simulink model "TEPC_Electronics"  (R2025a)
settings: Solver=FixedStepDiscrete  StartTime=0.0  StopTime=Inf  FixedStep=TEPC_Ts  RelTol=1e-3
undefined symbols (not defined in the file): TEPC_denCR, TEPC_denCSAPZ, TEPC_denRC, TEPC_numCR, TEPC_numCSAPZ, TEPC_numRC, TEPC_thrOff, TEPC_thrOn, TEPC_Ts
settings Model: Creator=ZWS  LastModifiedBy=ZWS

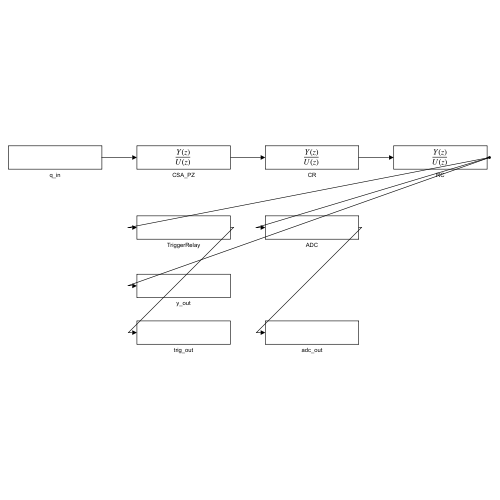
[thumbnail: Simulink's stored preview of the top-level diagram]
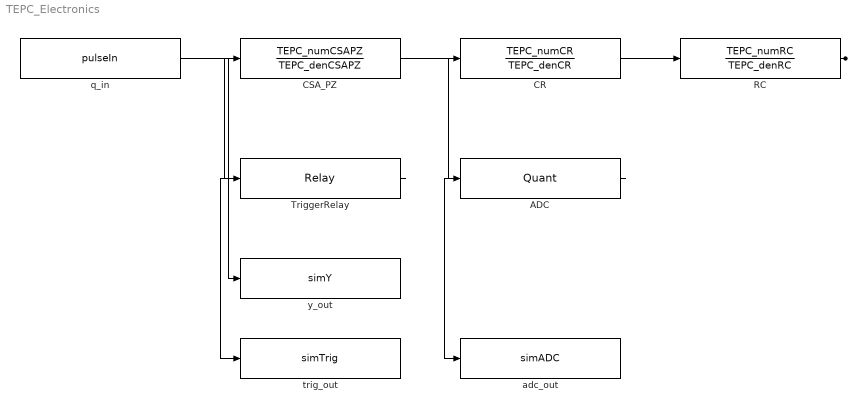
== system TEPC_Electronics ==
  ADC : Quantizer  QuantizationInterval=TEPC_lsb  SampleTime=TEPC_Ts
  CR : DiscreteTransferFcn  Numerator=TEPC_numCR  Denominator=TEPC_denCR  SampleTime=TEPC_Ts
  CSA_PZ : DiscreteTransferFcn  Numerator=TEPC_numCSAPZ  Denominator=TEPC_denCSAPZ  SampleTime=TEPC_Ts
  RC : DiscreteTransferFcn  Numerator=TEPC_numRC  Denominator=TEPC_denRC  SampleTime=TEPC_Ts
  TriggerRelay : Relay  OnSwitchValue=TEPC_thrOn  OffSwitchValue=TEPC_thrOff
  adc_out : ToWorkspace  VariableName=simADC  SampleTime=-1
  q_in : FromWorkspace  VariableName=pulseIn  SampleTime=TEPC_Ts
  trig_out : ToWorkspace  VariableName=simTrig  SampleTime=-1
  y_out : ToWorkspace  VariableName=simY  SampleTime=-1
  wires:
  q_in/1 -> CSA_PZ/1
  CSA_PZ/1 -> CR/1
  CR/1 -> RC/1
  RC/1 -> y_out/1, TriggerRelay/1, ADC/1
  TriggerRelay/1 -> trig_out/1
  ADC/1 -> adc_out/1
